simulink model "powertrain_model"  (R2025a)
settings: Solver=ode23tb  StartTime=0.0  StopTime=simlength  FixedStep=tc  MaxStep=tc
values from neighbouring files (symbols this model uses):
  angle_error = angle_error_deg/180*pi    (= 0)    [init_model.m]
  CTRPIFF_CLIP_RELEASE = 0.001    [init_model.m]
  dead_time = dead_time_INV    (= 4.2e-07)    [init_model.m]
  dead_time_INV = 0.42e-6    (= 4.2e-07)    [init_model.m]
  DThs_init = 0    [init_model.m]
  emf_fb_p = 0.2    [init_model.m]
  emf_fb_p_ccaller_1 = emf_fb_p    (= 0.2)    [init_model.m]
  emf_fb_p_ccaller_2 = emf_fb_p    (= 0.2)    [init_model.m]
  emf_p = emf_fb_p*4/10    (= 0.08)    [init_model.m]
  emf_p_ccaller_1 = emf_fb_p_ccaller_1*4/10    (= 0.08)    [init_model.m]
  emf_p_ccaller_2 = emf_fb_p_ccaller_2*4/10    (= 0.08)    [init_model.m]
  fPWM_INV = 25e3    (= 25000)    [init_model.m]
  g0_reference_flt = fcut_reference_flt * ts_inv * 2*pi    (= 0.00100530964915)    [init_model.m]
  g1_reference_flt = 1 - g0_reference_flt    (= 0.998994690351)    [init_model.m]
  id_ref_if_pu = iload_rms_ref*sqrt(2)/ibez    [init_model.m]
  kalman_omega = kw    [init_model.m]
  kalman_theta = kg    [init_model.m]
  kg = K(1)    [init_model.m]
  ki_id = 2    [analysis_cc.m]    (also in init_model.m = 9)
  ki_iq = 9    [init_model.m]
  ki_w = 1    [init_model.m]
  kp_id = 0.15    [analysis_cc.m]    (also in init_model.m = 0.25)
  kp_iq = 0.2    [init_model.m]
  kp_w = 1    [init_model.m]
  kw = K(2)    [init_model.m]
  luenberger_l1 = Klo(1)    [init_model.m]
  luenberger_l2 = Klo(2)    [init_model.m]
  luenberger_l3 = Klo(3)    [init_model.m]
  motorc_m_scale = 2/3*Vdc_bez/ubez    [init_model.m]
  number_of_cells = 100    [init_model.m]
  omega_flt_fcut = 10    [init_model.m]
  omega_flt_g0 = omega_flt_fcut * ts_inv * 2*pi    (= 0.00251327412287)    [init_model.m]
  omega_flt_g1 = 1 - omega_flt_g0    (= 0.997486725877)    [init_model.m]
  omega_ref_if_pu = 1200*2*pi/omega_bez    [init_model.m]
  phase_compensation_omega = 0    [init_model.m]
  pwm_out_lim = 1    [init_model.m]
  Q = 10    [init_model.m]
  q1Kalman = ts_inv^2    (= 1.6e-09)    [init_model.m]
  q2Kalman = ts_inv^1    (= 4e-05)    [init_model.m]
  q3Kalman = 0    [init_model.m]
  rKalman = 1    [init_model.m]
  Tambient = 1    [init_model.m]
  tc = ts_inv/200    (= 2e-07)    [init_model.m]
  time_init = 0.025    [init_model.m]
  torque_ref = 64/ibez*torque_mode    [init_model.m]
  ts_inv = 1/fPWM_INV    (= 4e-05)    [init_model.m]
  tsample = ts_inv    (= 4e-05)    [init_model.m]
  u_flt_g0 = u_flt_fcut * ts_inv * 2*pi    (= 0.904778684234)    [init_model.m]
  u_flt_g1 = 1 - u_flt_g0    (= 0.0952213157661)    [init_model.m]
  Vdc_bez = 400    [init_model.m]
undefined symbols (not defined in the file or in its folder): b, ibez, Jm, Jm_norm, Ld_norm, Lq_norm, Ls_norm, magnitude, omega_bez, psi_bez, psi_m, psi_m_norm, R_RLload, Rload_eq, Rs_norm, tau_bez, weigth
libraries: fl_lib x100, nesl_utility x84, ee_lib x11, cstblocks x4, lithium_ion_cell_lib x1, simulink x1, pmsm_uvw_with_harmonics_lib x1, pmsm_spatial_harmonics_uvw_lib x1, flexshaft_lib x1
(part 6 of 6)

== matlab function powertrain_model/inverter/MOS based inverter/threePhsModulator/uvw2alphabeta1 ==
  data: alpha input; u output; beta input; v output; w output
function [u,v,w] = alphabeta2uvw(alpha,beta)

u  = alpha;
v  = -0.5*alpha+sqrt(3)/2*beta;
w  = -0.5*alpha-sqrt(3)/2*beta;

end
